simulink model "dcdc_buffer"  (R2026a)
settings: Solver=ode23tb  StopTime=simlength  FixedStep=tc  MaxStep=glb_time.tc
values from neighbouring files (symbols this model uses):
  afe_ctrl = ctrl_afe_setup(glb_time.ts_afe, grid_emu.omega_grid_nom)    [init_model_legacy.m]
  frequency_set = 300    [init_model_legacy.m]
  glb_time = timing_setup(fpwm_afe, trgo_afe, fpwm_inv, trgo_inv, fpwm_single_phase_inv, trgo_single_phase_inv, fpwm_dab, trgo_dab,      fpwm_psfbc, trgo_psfbc, fpwm_isop_rail, trgo_isop_rail, fpwm_cllc, trgo_cllc, t_measure, tc_factor, tc_decimation, delay_pwm, dead_time_afe,      dead_time_inv, dead_time_single_phase_inv, dead_time_dab, dead_time_psfbc, dead_time_isop_rail, dead_time_cllc)    [init_model_legacy.m]
  grid_emu = grid_three_phase_emulator('Dyn11', delta_star, grid_nominal_power, application_voltage, us1, us2, fgrid,                  eq_grid_inductance, eq_grid_resistance, eta, ucc, i1m, p_iron, n1, n2, core_area, core_length, mur,                  up_xi_pu_ref, up_eta_pu_ref, un_xi_pu_ref, un_eta_pu_ref)    [init_model_legacy.m]
  heatsink = liquid_cooled_plate_2kw_setup(weight, no_weight, cp_al, heat_capacity_hs, thermal_conductivity_al,      Rth_switch_HA, Rth_mosfet_HA, Rth_diode_HA, Tambient, DThs_init)    [init_model_legacy.m]
  Tambient = 40    [init_model_legacy.m]
undefined symbols (not defined in the file or in its folder): hwdata, igbt, magnitude
libraries: fl_lib x113, nesl_utility x63, igbt_simple_2th_lib x4, ee_lib x2, pi_ctrl x2, dq_vector_pi x1, linear_double_integrator_observer_ccaller x1, phase_shift_filter_ccaller x1, discrete_time_low_pass_filter x1, single_phase_pwm_modulator x1, three_phase_voltage_with_frt_emulator x1
(part 4 of 4)

== system dcdc_buffer/dclink_voltage_cmp/dclink_cmp/dclink_compensation_ctrl/grid_phase_pll/FHT-PLL/pll_stageA/filter_and_transformation/FHTbeta ==
  u : Inport
  Bus Selector : BusSelector  OutputSignals=output_pu_hat,output_pu_hat_dot
  C Caller : CCaller  FunctionName=first_harmonic_tracker_process_simulink  PortSpecificationStruct="%)30     .    B \\   8    (     @         %    \"     D    !     0         %  0 \"0    $    _    07)G3F%M90  4&]R=$YA;64 4V-O<&4     26YD97@     5'EP90      4VEZ90      27-';&]B86P   X    P    !@    @    $          4    (     0    ,    !         !   P!O=70 #@   #     &    \"     0         !0    @    !     P    $         $  # &]U=  .    .     8    (    !          %    \"     $    &     0         0  ...(+4988 chars)"
  Constant : Constant  Value=glb_time.ts_afe
  Constant1 : Constant  Value=2
  Constant4 : Constant  Value=afe_ctrl.fht_grid.omega_fht
  Constant5 : Constant  Value=afe_ctrl.fht_grid.delta_fht
  Constant6 : Constant  Value=afe_ctrl.fht_grid.Ld_fht(1)
  Constant7 : Constant  Value=afe_ctrl.fht_grid.Ld_fht(2)
  Data Type Conversion{1..2,6..9} (6 alike) : DataTypeConversion  OutDataTypeStr=single  SaturateOnIntegerOverflow=off  RndMeth=Floor
  Data Type Conversion10 : DataTypeConversion  OutDataTypeStr=double  SaturateOnIntegerOverflow=off  RndMeth=Floor
  Data Type Conversion3 : DataTypeConversion  OutDataTypeStr=uint8  SaturateOnIntegerOverflow=off  RndMeth=Floor
  Data Type Conversion4 : DataTypeConversion  OutDataTypeStr=double  SaturateOnIntegerOverflow=off  RndMeth=Floor
  Data Type Conversion5 : DataTypeConversion  OutDataTypeStr=uint8  SaturateOnIntegerOverflow=off  RndMeth=Floor
  Gain : Gain  Gain=1/afe_ctrl.fht_grid.omega_fht
  Step : Step  Time=0.0125  InitialValue=1  FinalValue=0
  ud_hat : Outport
  uq_hat : Outport  Port=2
  wires:
  Gain/1 -> uq_hat/1
  Bus Selector/2 -> Data Type Conversion10/1  "<output_pu_hat_dot>"
  Data Type Conversion10/1 -> Gain/1
  Data Type Conversion4/1 -> ud_hat/1
  Data Type Conversion3/1 -> C Caller/1
  Data Type Conversion1/1 -> C Caller/3
  Data Type Conversion2/1 -> C Caller/2
  C Caller/1 -> Bus Selector/1
  Bus Selector/1 -> Data Type Conversion4/1  "<output_pu_hat>"
  Step/1 -> Data Type Conversion3/1
  u/1 -> Data Type Conversion2/1
  Constant/1 -> Data Type Conversion1/1
  Constant1/1 -> Data Type Conversion5/1
  Constant4/1 -> Data Type Conversion6/1
  Constant6/1 -> Data Type Conversion8/1
  Constant7/1 -> Data Type Conversion9/1
  Constant5/1 -> Data Type Conversion7/1
  Data Type Conversion5/1 -> C Caller/8
  Data Type Conversion6/1 -> C Caller/4
  Data Type Conversion7/1 -> C Caller/5
  Data Type Conversion8/1 -> C Caller/6
  Data Type Conversion9/1 -> C Caller/7

== matlab function dcdc_buffer/dclink_voltage_cmp/dclink_cmp/dclink_compensation_ctrl/grid_phase_pll/FHT-PLL/pll_stageA/filter_and_transformation/abc2alphabeta ==
  data: a input; alpha output; b input; c input; beta output
function [alpha,beta] = abc2alphabeta(a,b,c)

alpha = 2/3*(a - 1/2*b - 1/2*c);
beta  = 1/sqrt(3)*(b - c);

end

== matlab function dcdc_buffer/dclink_voltage_cmp/dclink_cmp/dclink_compensation_ctrl/grid_phase_pll/FHT-PLL/pll_stageB/bounder1 ==
  data: u input; y output
function y = bounder(u)
    y = -pi + mod(u+3*pi,2*pi);
end

== matlab function dcdc_buffer/dclink_voltage_cmp/dclink_cmp/dclink_compensation_ctrl/grid_phase_pll/FHT-PLL/pll_stageA/sequences/alphabeta2xieta ==
  data: alpha input; xi output; beta input; gamma input; eta output
function [xi,eta] = alphabeta2xieta_pos(alpha,beta,gamma)

    xi  =  (alpha*cos(gamma) + beta*sin(gamma));
    eta = (-alpha*sin(gamma) + beta*cos(gamma));

end

== matlab function dcdc_buffer/dclink_voltage_cmp/dclink_cmp/dclink_compensation_ctrl/grid_phase_pll/FHT-PLL/pll_stageB/double_integrator_observer/bounder1 ==
  data: u input; y output
function y = bounder(u)
    
    y = -pi + mod(u+3*pi,2*pi);
    
end

== matlab function dcdc_buffer/dclink_voltage_cmp/dclink_cmp/dclink_compensation_ctrl/dclink_ripple_compensation_rpi/alphabeta2dq/MATLAB Function ==
  data: alpha input; d output; beta input; phase input; q output
function [d, q] = alphabeta2dq(alpha, beta, phase)

d = alpha*cos(phase) + beta*sin(phase);
q = -alpha*sin(phase) + beta*cos(phase);

== matlab function dcdc_buffer/dclink_voltage_cmp/dclink_cmp/dclink_compensation_ctrl/dclink_ripple_compensation_rpi/dq2alphabeta/MATLAB Function ==
  data: d input; alpha output; q input; phase input; beta output
function [alpha, beta] = dq2alphabeta(d, q, phase)

alpha = d*cos(phase) - q*sin(phase);
beta = d*sin(phase) + q*cos(phase);

== matlab function dcdc_buffer/dclink_voltage_cmp/dclink_cmp/dclink_compensation_ctrl/grid_phase_pll/FHT-PLL/pll_stageB/double_integrator_observer/bounder2 ==
  data: u input; y output
function y = bounder(u)
    
    y = -pi + mod(u+3*pi,2*pi);
    
end
